simulink model "pd_to_wheel_1"  (R2026a)
settings: Solver=ode45  StopTime=200  MaxStep=0.1
settings Model: Creator=user  LastModifiedBy=user

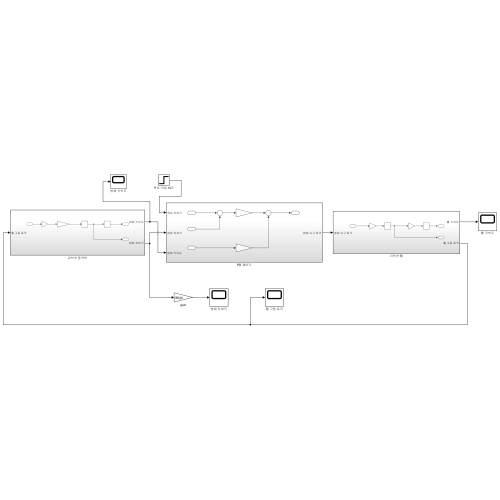
[thumbnail: Simulink's stored preview of the top-level diagram]
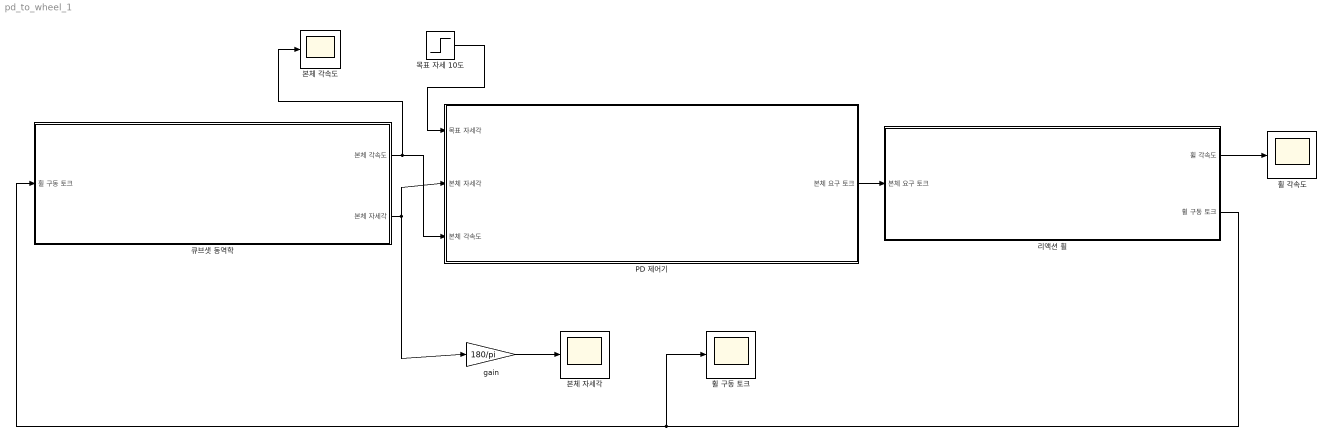
== system pd_to_wheel_1 ==
  PD 제어기 : Subsystem
  gain : Gain  Gain=180/pi
  리액션 휠 : Subsystem
  목표 자세 10도 : Step  FinalValue=10*pi/180  SampleTime=0
  본체 각속도 : Scope
      settings: ActiveDisplayYMinimum=-0.0017027849116373866  ActiveDisplayYMaximum=0.013283712334869111  DataLoggingVariableName=ScopeData2
  본체 자세각 : Scope
      settings: ActiveDisplayYMinimum=-1.2716519027276829  ActiveDisplayYMaximum=11.444867124549148
  큐브샛 동역학 : Subsystem
  휠 각속도 : Scope
      settings: ActiveDisplayYMinimum=-120.7610212260828  ActiveDisplayYMaximum=15.479862833067092
  휠 구동 토크 : Scope
      settings: ActiveDisplayYMinimum=-0.00040065675177193073  ActiveDisplayYMaximum=0.00011525226195871713  DataLoggingVariableName=ScopeData3
  wires:
  PD 제어기/1(본체 요구 토크) -> 리액션 휠/1(본체 요구 토크)
  큐브샛 동역학/1(본체 각속도) -> 본체 각속도/1, PD 제어기/3(본체 각속도)
  큐브샛 동역학/2(본체 자세각) -> PD 제어기/2(본체 자세각), gain/1
  리액션 휠/2(휠 구동 토크) -> 큐브샛 동역학/1(휠 구동 토크), 휠 구동 토크/1
  목표 자세 10도/1 -> PD 제어기/1(목표 자세각)
  리액션 휠/1(휠 각속도) -> 휠 각속도/1
  gain/1 -> 본체 자세각/1

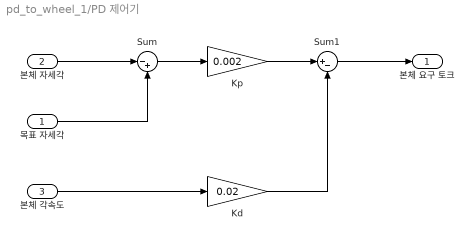
== system pd_to_wheel_1/PD 제어기 ==
  목표 자세각 : Inport
  본체 자세각 : Inport  Port=2
  본체 각속도 : Inport  Port=3
  Kd : Gain  Gain=0.02
  Kp : Gain  Gain=0.002
  Sum : Sum  Inputs=|-+
  Sum1 : Sum  Inputs=|+-
  본체 요구 토크 : Outport
  wires:
  본체 자세각/1 -> Sum/1
  Kd/1 -> Sum1/2
  Kp/1 -> Sum1/1
  본체 각속도/1 -> Kd/1
  Sum1/1 -> 본체 요구 토크/1
  Sum/1 -> Kp/1
  목표 자세각/1 -> Sum/2

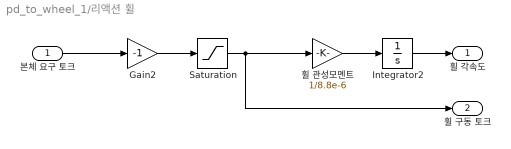
== system pd_to_wheel_1/리액션 휠 ==
  본체 요구 토크 : Inport
  Gain2 : Gain  Gain=-1
  Integrator2 : Integrator
  Saturation : Saturate  UpperLimit=0.001  LowerLimit=-0.001
  휠 관성모멘트 : Gain  Gain=1/8.8e-6
  휠 각속도 : Outport
  휠 구동 토크 : Outport  Port=2
  wires:
  본체 요구 토크/1 -> Gain2/1
  Integrator2/1 -> 휠 각속도/1
  휠 관성모멘트/1 -> Integrator2/1
  Gain2/1 -> Saturation/1
  Saturation/1 -> 휠 관성모멘트/1, 휠 구동 토크/1

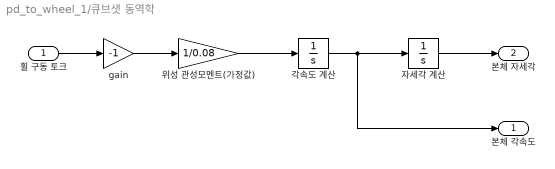
== system pd_to_wheel_1/큐브샛 동역학 ==
  휠 구동 토크 : Inport
  gain : Gain  Gain=-1
  각속도 계산 : Integrator
  위성 관성모멘트(가정값) : Gain  Gain=1/0.08
  자세각 계산 : Integrator
  본체 각속도 : Outport
  본체 자세각 : Outport  Port=2
  wires:
  위성 관성모멘트(가정값)/1 -> 각속도 계산/1
  gain/1 -> 위성 관성모멘트(가정값)/1
  각속도 계산/1 -> 본체 각속도/1, 자세각 계산/1
  휠 구동 토크/1 -> gain/1
  자세각 계산/1 -> 본체 자세각/1
